simulink model "systeme_complet"  (R2022b)
settings: Solver=FixedStepAuto  StartTime=0.0  StopTime=t_stop  FixedStep=Ts  RelTol=1e-3
InitFcn:
  | parametres
undefined symbols (not defined in the file): f_dec, f_out, I_ref, Ki, Kp, M_ref, R_ch, Ts
libraries: fl_lib x22, ee_lib x18, nesl_utility x17, simulink x2, slpidlib x1
settings Model: Creator=HP  LastModifiedBy=HP

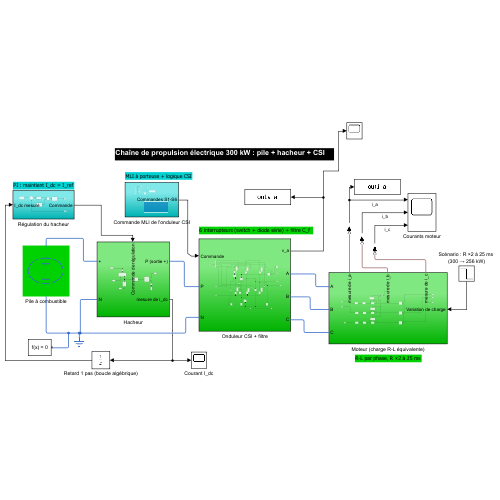
[thumbnail: Simulink's stored preview of the top-level diagram]
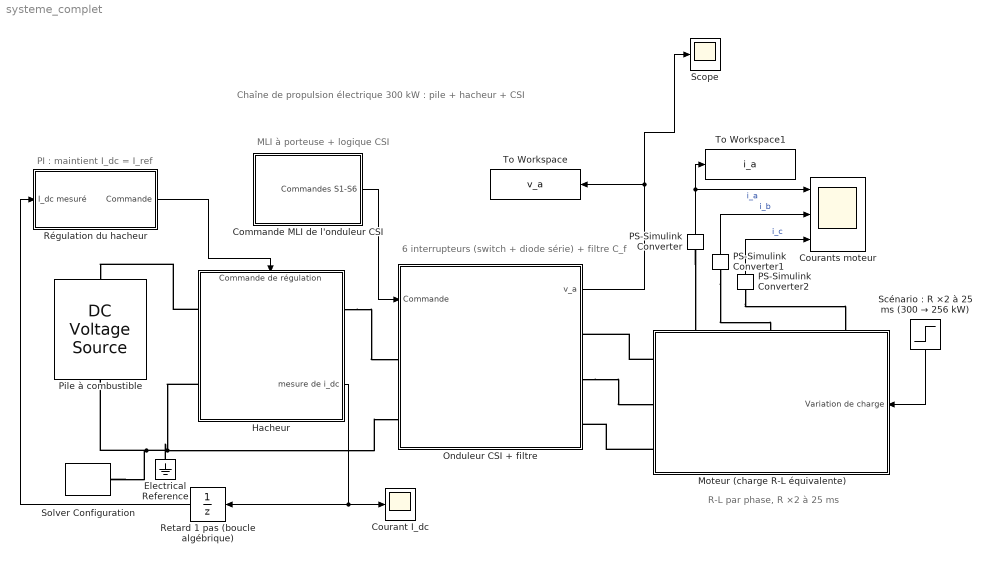
== system systeme_complet ==
  note: R-L par phase, R ×2 à 25 ms
  note: 6 interrupteurs (switch + diode série) + filtre C_f
  note: MLI à porteuse + logique CSI
  note: PI : maintient I_dc = I_ref
  note: Chaîne de propulsion électrique 300 kW : pile + hacheur + CSI
  Commande MLI de l'onduleur CSI : Subsystem
  Courant I_dc : Scope
  Courants moteur : Scope  NumInputPorts=3
  Electrical Reference : fl_lib/Electrical/Electrical Elements/Electrical Reference
  Hacheur : Subsystem
      settings: PortSchema="{\"entries\":[{\"content\":{\"sides\":[{\"content\":{\"connectorIds\":[\"LConn1\",\"LConn2\"]},\"type\":\"ConnectorPlacement.EquallySpacedRectSide\",\"uuid\":\"2dac1032-4ca4-4438-a519-692aa5ca1595\"},{\"content\":{\"connectorIds\":[\"RConn1\",\"Out1\"],\"side\":\"RIGHT\"},\"type\":\"ConnectorPlacement.EquallySpacedRectSide\",\"uuid\":\"94db1daf-747a-46bc-a51a-2b17978c1da3\"},{\"content\":{\"connectorIds\":[\"In1\"],\"side\":\"TOP\"},\"type\":\"ConnectorPlacement.EquallySpacedRectSide\",\"uuid\":\"3d1b3b24-76d5-4cf6-b9a4-916d1a1a4593\"},{\"content\":{\"connectorIds\":[],\"side\":\"BOTTOM\"},\"type\":\"ConnectorPlacement.EquallySpacedRectSide\",\"uuid\":\"3f80dfdd-caf6-41fc-aca6-59b801a18497\"}]},\"type\":\"ConnectorPlacement.EquallySpacedConnector\",\"uuid\":\"7bb300ac-b427-4bc8-9636-bf9acc93662d\"}],\"packageUris\":[\"http://schema.mathworks.com/mf0/Connector/R2020b\"],\"version\":\"1.0\"}"
  Moteur (charge R-L équivalente) : Subsystem
      settings: PortSchema="{\"entries\":[{\"content\":{\"sides\":[{\"content\":{\"connectorIds\":[\"LConn1\",\"LConn2\",\"LConn3\"]},\"type\":\"ConnectorPlacement.EquallySpacedRectSide\",\"uuid\":\"3a5aebfa-ac8c-4dc1-bdc7-0f42fa247e71\"},{\"content\":{\"connectorIds\":[\"In1\"],\"side\":\"RIGHT\"},\"type\":\"ConnectorPlacement.EquallySpacedRectSide\",\"uuid\":\"61d8263a-5991-459d-931c-dea362971dfc\"},{\"content\":{\"connectorIds\":[\"LConn4\",\"LConn5\",\"LConn6\"],\"side\":\"TOP\"},\"type\":\"ConnectorPlacement.EquallySpacedRectSide\",\"uuid\":\"dbe65e42-3578-4df4-96b5-9b98adcff1b2\"}]},\"type\":\"ConnectorPlacement.EquallySpacedConnector\",\"uuid\":\"a1fde088-52d3-4f5b-92ff-46a317a2fe9e\"}],\"packageUris\":[\"http://schema.mathworks.com/mf0/Connector/R2020b\"],\"version\":\"1.0\"}"
  Onduleur CSI + filtre : Subsystem
  PS-Simulink Converter : nesl_utility/PS-Simulink Converter  PhysicalDomain=network_engine_domain  SubClassName=ps_output  LeftPortType=input  RightPortType=output  PseudoPeriodic=off  Frequencies=[]  VectorFormat=inherit  Unit=A  AffineConversion=off
  PS-Simulink Converter1 : nesl_utility/PS-Simulink Converter  PhysicalDomain=network_engine_domain  SubClassName=ps_output  LeftPortType=input  RightPortType=output  PseudoPeriodic=off  Frequencies=[]  VectorFormat=inherit  Unit=A  AffineConversion=off
  PS-Simulink Converter2 : nesl_utility/PS-Simulink Converter  PhysicalDomain=network_engine_domain  SubClassName=ps_output  LeftPortType=input  RightPortType=output  PseudoPeriodic=off  Frequencies=[]  VectorFormat=inherit  Unit=A  AffineConversion=off
  Pile à combustible : fl_lib/Electrical/Electrical Sources/DC Voltage Source  v0=V_pile V
  Retard 1 pas (boucle algébrique) : UnitDelay  SampleTime=-1  HasFrameUpgradeWarning=on
  Régulation du hacheur : Subsystem
  Scope : Scope
  "Scénario : R ×2 à 25 ms (300 → 256 kW)" : Step  Time=0.025  Before=1  After=0  SampleTime=0
  Solver Configuration : nesl_utility/Solver Configuration  PhysicalDomain=network_engine_domain  SubClassName=solver  LeftPortType=input  RightPortType=generic  Tones=[]  Harmonics=[]  SimulateNoise=off  Profile=off  UseLocalSampling=off  EnableSwitchedLinearOptims=on  FrequencyDomain=off  UseCCode=off  RelTol=0.001  AbsTol=0.001  MinStep=1e-09  ToWorkspace=off  RevertToSquareIcSolve=off  NumHomotopyIterations=100  PhasorMode=off  PhasorModeNumHarmonics=1  ConsistencySolver=NEWTON_XTOL_AFTER_FTOL  IndexReductionMethod=DerivativeReplacement  DoDC=off  ResidualTolerance=1e-09  ConsistencyTolSource=GLOBAL  ConsistencyAbsTol=0.001  ConsistencyRelTol=0.001  ConsistencyTolFactor=0.001  UseLocalSolver=on  LocalSolverChoice=NE_PARTITIONING_ADVANCER  ResolveIndetEquations=on  FunctionEvalNumThread=1  LocalSolverSampleTime=Ts  DoFixedCost=on  MaxNonlinIter=3  MaxModeIter=2  ComputeImpulses=off  ImpulseIterations=2  LinearAlgebra=auto  LinearAlgebraNumThread=0  EquationFormulation=NE_TIME_EF  DelaysMemoryBudget=1024  AutomaticFiltering=on  FilteringTimeConstant=0.001  PartitionStorageMethod=AS_NEEDED  PartitionMemoryBudget=1024  PartitionMethod=ROBUST
  To Workspace : ToWorkspace  VariableName=v_a  SaveFormat=Timeseries  SampleTime=Ts
  To Workspace1 : ToWorkspace  VariableName=i_a  SaveFormat=Timeseries  SampleTime=Ts
  wires:
  PS-Simulink Converter/1 -> Courants moteur/1, To Workspace1/1  "i_a"
  PS-Simulink Converter1/1 -> Courants moteur/2  "i_b"
  PS-Simulink Converter2/1 -> Courants moteur/3  "i_c"
  Hacheur/1(mesure de i_dc) -> Retard 1 pas (boucle algébrique)/1, Courant I_dc/1
  "Scénario : R ×2 à 25 ms (300 → 256 kW)"/1 -> Moteur (charge R-L équivalente)/1(Variation de charge)
  Retard 1 pas (boucle algébrique)/1 -> Régulation du hacheur/1(I_dc mesuré)
  Régulation du hacheur/1(Commande) -> Hacheur/1(Commande de régulation)
  Commande MLI de l'onduleur CSI/1(Commandes S1-S6) -> Onduleur CSI + filtre/1(Commande)
  Onduleur CSI + filtre/1(v_a) -> Scope/1, To Workspace/1
  connections:
  Hacheur/LConn1 -- Pile à combustible/LConn1
  Hacheur/LConn2 -- Electrical Reference/LConn1 -- Pile à combustible/RConn1 -- Solver Configuration/RConn1 -- Onduleur CSI + filtre/LConn2
  PS-Simulink Converter/LConn1 -- Moteur (charge R-L équivalente)/LConn4
  PS-Simulink Converter1/LConn1 -- Moteur (charge R-L équivalente)/LConn5
  PS-Simulink Converter2/LConn1 -- Moteur (charge R-L équivalente)/LConn6
  Hacheur/RConn1 -- Onduleur CSI + filtre/LConn1
  Moteur (charge R-L équivalente)/LConn3 -- Onduleur CSI + filtre/RConn3
  Moteur (charge R-L équivalente)/LConn1 -- Onduleur CSI + filtre/RConn1
  Onduleur CSI + filtre/RConn2 -- Moteur (charge R-L équivalente)/LConn2

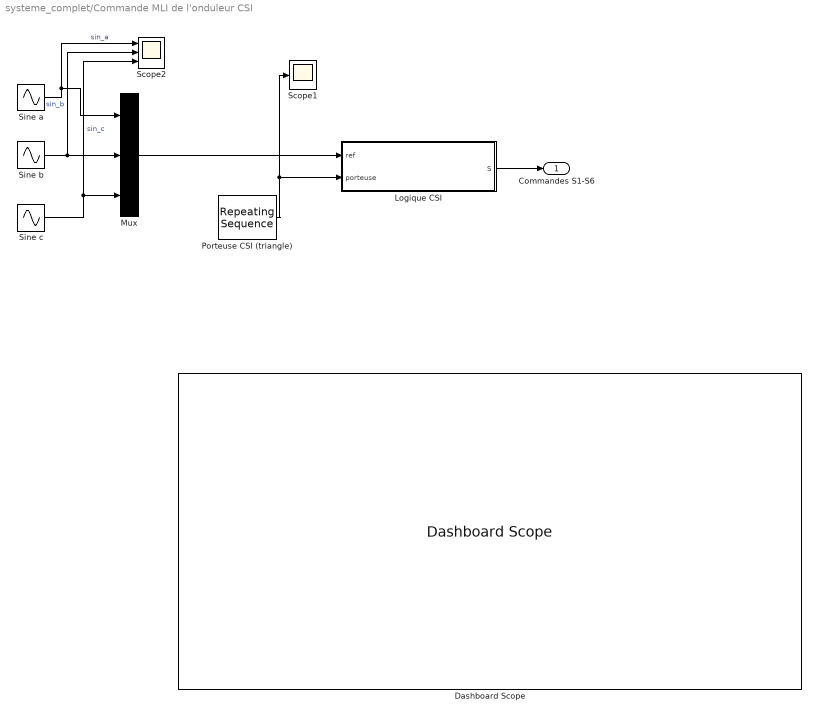
== system systeme_complet/Commande MLI de l'onduleur CSI ==
  Dashboard Scope : DashboardScope
  Logique CSI : MATLAB Function  TreatAsAtomicUnit=on
  Mux : Mux  Inputs=3
  Porteuse CSI (triangle) : simulink/Sources/Repeating Sequence  rep_seq_t=[0 1/(2*f_dec) 1/f_dec]  rep_seq_y=[-1 1 -1]
  Scope1 : Scope
  Scope2 : Scope  NumInputPorts=3
  Sine a : Sin  Amplitude=M_ref  Frequency=2*pi*f_out  SampleTime=Ts
  Sine b : Sin  Amplitude=M_ref  Frequency=2*pi*f_out  Phase=-2*pi/3  SampleTime=Ts
  Sine c : Sin  Amplitude=M_ref  Frequency=2*pi*f_out  Phase=2*pi/3  SampleTime=Ts
  Commandes S1-S6 : Outport
  wires:
  Logique CSI/1(S) -> Commandes S1-S6/1
  Sine b/1 -> Scope2/2, Mux/2  "sin_b"
  Sine c/1 -> Scope2/3, Mux/3  "sin_c"
  Mux/1 -> Logique CSI/1(ref)
  Sine a/1 -> Scope2/1, Mux/1  "sin_a"
  Porteuse CSI (triangle)/1 -> Scope1/1, Logique CSI/2(porteuse)

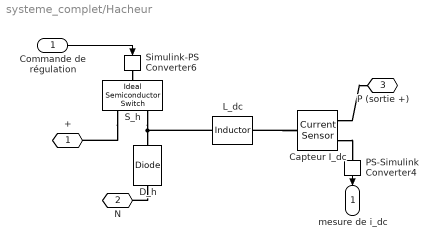
== system systeme_complet/Hacheur ==
  Commande de régulation : Inport
  Capteur I_dc : fl_lib/Electrical/Electrical Sensors/Current Sensor
  D_h : ee_lib/Semiconductors & Converters/Diode  ModelType=ee.enum.diode.modelType.pwl  TableType=ee.enum.diode.tableType.IfMat  IfMat=[.07, .12, .19, 1.75, 4.24, 7.32, 11.2; .16, .3, .72, 2.14, 5.02, 8.35, 13.12] A  VfMat=[.9, 1.15, 1.25, 1.5, 1.75, 2.17, 2.6, 2.85; .58, .68, .75, 1.1, 1.38, 1.77, 2.27, 2.7] V  TjVec=[25, 125] degC  VfVec=[.5, .7, .9, 1.3, 1.7, 2.1, 2.5] V  IfVec=[.1, .2, .5, 1, 2, 4, 7, 10] A  Vf=V_f V  Ron=R_on Ohm  Goff=G_off S  prmExp=ee.enum.diode.expParam.useTwo  I12=[.0137, .545] A  V12=[.6, .7] V  RS=0 Ohm  Tmeas=25 degC  IS=1e-12 A  ec=1  I1=0.0137 A  V1=0.6 V  N_series=1  N_parallel=1  Rz=0.3 Ohm  BV=inf V  C_param=ee.enum.diode.capParam.fixed  CJ=0 pF  CJ0=5 pF  Vvec=[.1, 10, 100] V  Cvec=[3.5, 1, .4] pF  VJ=1 V  Mgrad=0.5  FC=0.5  Q_param=ee.enum.diode.recoveryParam.off  iRM=-7.15 A  iF=4 A  didt=-750 A/us  trr_factor=3  trr=115 ns  Qrr=150 nA*s  Vr=-600 V  Ls=150 nH  Erec=0.03 J  TT=50 ns  tau=100 ns  T_param=ee.enum.diode.temperatureParam.off  Tdevice=25 degC  I1_T2=0.245 A  V1_T2=0.5 V  IS_T2=1.25e-7 A  Tmeas2=125 degC  XTI_param=ee.enum.diode.xtiParam.pn  XTI=3  EG_param=ee.enum.diode.egapParam.material_si  EG=1.11 eV  dBVdT=0 V/K  enable_faults=simscape.enum.onoff.off  fault_action=simscape.enum.assert.action.none  fault_types=ee.enum.diode.faults.open  tau_fault=1e-3 s  IfMat_faulted=[.07, .12, .19, 1.75, 4.24, 7.32, 11.2; .16, .3, .72, 2.14, 4.02, 6.35, 9.12] A  VfMat_faulted=[.9, 1.15, 1.25, 1.5, 1.75, 2.17, 2.6, 2.85; .58, .68, .75, 1.1, 1.38, 1.77, 2.27, 2.7] V  VfVec_faulted=[.5, .7, .9, 1.3, 1.7, 2.1, 2.5] V  IfVec_faulted=[.1, .2, .5, 1, 2, 4, 7, 10] A  Ropen_faulted=1000 Ohm  Gshort_faulted=1000 1/Ohm  Vf_faulted=0.6 V  Ron_faulted=0.3 Ohm  Goff_faulted=1e-8 S  I12_faulted=[.0137, .545] A  V12_faulted=[.6, .7] V  IS_faulted=1e-12 A  ec_faulted=1  I1_faulted=0.0137 A  V1_faulted=0.6 V  RS_faulted=0 Ohm  Rz_faulted=0.3 Ohm  BV_faulted=inf V  Cscale_faulted=100  enable_temporal_fault=simscape.enum.onoff.off  t_fault=inf s  enable_behavioral_fault=simscape.enum.onoff.off  max_permissible_voltage=inf V  n_fail_on_voltage=1  max_permissible_current=inf A  t_fail_on_current=1 s  max_permissible_dVdt=inf V/s  enable_fault_input=simscape.enum.onoff.off  i_specify=off  i_priority=None  i=0 A  i_nominal_specify=off  i_nominal_unit=A  i_nominal_value=1  v_specify=off  v_priority=None  v=0 V  v_nominal_specify=off  v_nominal_unit=V  v_nominal_value=1  v_capacitor_specify=off  v_capacitor_priority=None  v_capacitor=0 V  v_capacitor_nominal_specify=off  v_capacitor_nominal_unit=V  v_capacitor_nominal_value=1  i_diode_specify=off  i_diode_priority=None  i_diode=0 A  i_diode_nominal_specify=off  i_diode_nominal_unit=A  i_diode_nominal_value=1  v_diode_specify=off  v_diode_priority=None  v_diode=0 V  v_diode_nominal_specify=off  v_diode_nominal_unit=V  v_diode_nominal_value=1  i_capacitor_specify=off  i_capacitor_priority=None  i_capacitor=0 A  i_capacitor_nominal_specify=off  i_capacitor_nominal_unit=A  i_capacitor_nominal_value=1  power_dissipated_specify=off  power_dissipated_priority=None  power_dissipated=0 W  power_dissipated_nominal_specify=off  power_dissipated_nominal_unit=W  power_dissipated_nominal_value=1  fidelity_level=ee.enum.diode.fidelity.includeChargeDyn  rec_loss_model=ee.enum.diode.reverseRecoveryModel.fixed  ErecVal=0 J  ErecMat=zeros(2, 3) J  TjrecVec=[298.15, 398.15] K  IfrecVec=[.1, 1, 10] A  VrecVal=10 V  tFilter=1 / 1000 / 100 s  max_permissible_temperature=inf K  t_fail_on_temperature=1 s  thermal_network_parameterization=ee.enum.thermalNetworkTopology.junctionCase  Rth=[0, 10] K/W  Rth_Cauer=[1, 3, 10] K/W  Rth_Foster=[4, 6] K/W  thermal_mass_parameterization=ee.enum.thermalNetwork.timeconstant  thermal_mass=[0, 1] J/K  thermal_mass_Cauer=[.1, .3, 1] J/K  thermal_mass_Foster=[1.5, 3] J/K  thermal_time_constant=[0, 10] s  thermal_time_constant_Cauer=[1, 3, 10] s  thermal_time_constant_Foster=[6, 18] s  thermal_mass_initial_temperatures=[25, 25] degC  thermal_mass_initial_temperatures_Cauer=[25, 25, 25] degC  junction_thermal_mass=0.01 J/K  Tvec_initial_Foster=[25, 25, 25, 25] degC  no_thermal_network=0  junction_temperature_specify=off  junction_temperature_priority=None  junction_temperature=25 degC  junction_temperature_nominal_specify=off  junction_temperature_nominal_unit=degC  junction_temperature_nominal_value=1
  L_dc : ee_lib/Passive/Inductor  l=L_dc H  enable_L_tol=0  L_tol=20  tol_distribution=1  nSigma=4  r=0 Ohm  g=1e-9 1/Ohm  enable_operating_limits=0  operating_limit_action=2  max_working_current=1 A  power_rating=1 W  enable_faults=0  fault_action=1  lambdaPercent=50  k_faulted=0.9999  turnsShort=0  openCct=0  groundShort=0  groundShortG=0 1/Ohm  tau_fault=1e-3 s  enable_temporal_fault=0  t_fault=1 s  enable_behavioral_fault=0  max_permissible_voltage=100 V  n_fail_on_voltage=1  max_permissible_current=1 A  t_fail_on_current=1 s  i_L_specify=off  i_L_priority=High  i_L=0 A  i_L_nominal_specify=off  i_L_nominal_unit=A  i_L_nominal_value=1
  PS-Simulink Converter4 : nesl_utility/PS-Simulink Converter  PhysicalDomain=network_engine_domain  SubClassName=ps_output  LeftPortType=input  RightPortType=output  PseudoPeriodic=off  Frequencies=[]  VectorFormat=inherit  Unit=A  AffineConversion=off
  S_h : ee_lib/Semiconductors & Converters/Ideal Semiconductor Switch  port_option=ee.enum.controlport.ps  Ron=R_on Ohm  Goff=G_off 1/Ohm  Vth=0.5 V  diode_param=ee.enum.converters.protectiondiode.none  diode_Vf=0.8 V  diode_Ron=0.001 Ohm  diode_Goff=1e-5 1/Ohm  diode_C=50e-9 F  diode_iRM=-235 A  diode_iF=300 A  diode_idot=-50 A/us  diode_trr_param=ee.enum.converters.diodetrr.trr_factor  diode_trr_factor=3  diode_trr=15 us  diode_Qrr=1500 s*uA
  Simulink-PS Converter6 : nesl_utility/Simulink-PS Converter  PhysicalDomain=network_engine_domain  SubClassName=ps_input  LeftPortType=input  RightPortType=output  PseudoPeriodic=off  Frequencies=[]  NoiseDistribution=none  NoiseParameters=[]  Unit=1  AffineConversion=off  FilteringAndDerivatives=provide  SimscapeFilterOrder=1  InputFilterTimeConstant=0.001  UdotUserProvided=0
  + : PMIOPort  Side=Left
  N : PMIOPort  Port=2  Side=Left
  P (sortie +) : PMIOPort  Port=3  Side=Right
  mesure de i_dc : Outport
  wires:
  Commande de régulation/1 -> Simulink-PS Converter6/1
  PS-Simulink Converter4/1 -> mesure de i_dc/1
  connections:
  Capteur I_dc/LConn1 -- L_dc/RConn1
  Simulink-PS Converter6/RConn1 -- S_h/LConn1
  D_h/RConn1 -- S_h/RConn2 -- L_dc/LConn1
  S_h/RConn1 -- +/RConn1
  Capteur I_dc/RConn1 -- PS-Simulink Converter4/LConn1
  Capteur I_dc/RConn2 -- P (sortie +)/RConn1
  D_h/LConn1 -- N/RConn1

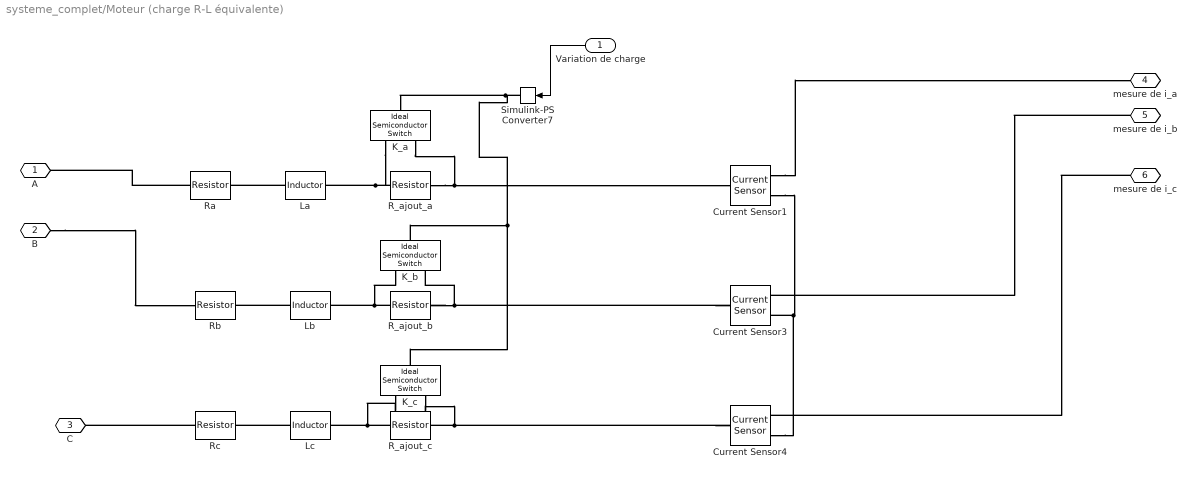
== system systeme_complet/Moteur (charge R-L équivalente) ==
  Variation de charge : Inport
  Current Sensor1 : fl_lib/Electrical/Electrical Sensors/Current Sensor
  Current Sensor3 : fl_lib/Electrical/Electrical Sensors/Current Sensor
  Current Sensor4 : fl_lib/Electrical/Electrical Sensors/Current Sensor
  K_a : ee_lib/Semiconductors & Converters/Ideal Semiconductor Switch  port_option=ee.enum.controlport.ps  Ron=R_on Ohm  Goff=G_off 1/Ohm  Vth=0.5 V  diode_param=ee.enum.converters.protectiondiode.none  diode_Vf=0.8 V  diode_Ron=0.001 Ohm  diode_Goff=1e-5 1/Ohm  diode_C=50e-9 F  diode_iRM=-235 A  diode_iF=300 A  diode_idot=-50 A/us  diode_trr_param=ee.enum.converters.diodetrr.trr_factor  diode_trr_factor=3  diode_trr=15 us  diode_Qrr=1500 s*uA
  K_b : ee_lib/Semiconductors & Converters/Ideal Semiconductor Switch  port_option=ee.enum.controlport.ps  Ron=R_on Ohm  Goff=G_off 1/Ohm  Vth=0.5 V  diode_param=ee.enum.converters.protectiondiode.none  diode_Vf=0.8 V  diode_Ron=0.001 Ohm  diode_Goff=1e-5 1/Ohm  diode_C=50e-9 F  diode_iRM=-235 A  diode_iF=300 A  diode_idot=-50 A/us  diode_trr_param=ee.enum.converters.diodetrr.trr_factor  diode_trr_factor=3  diode_trr=15 us  diode_Qrr=1500 s*uA
  K_c : ee_lib/Semiconductors & Converters/Ideal Semiconductor Switch  port_option=ee.enum.controlport.ps  Ron=R_on Ohm  Goff=G_off 1/Ohm  Vth=0.5 V  diode_param=ee.enum.converters.protectiondiode.none  diode_Vf=0.8 V  diode_Ron=0.001 Ohm  diode_Goff=1e-5 1/Ohm  diode_C=50e-9 F  diode_iRM=-235 A  diode_iF=300 A  diode_idot=-50 A/us  diode_trr_param=ee.enum.converters.diodetrr.trr_factor  diode_trr_factor=3  diode_trr=15 us  diode_Qrr=1500 s*uA
  La : fl_lib/Electrical/Electrical Elements/Inductor  l=L_ch H  r=0 Ohm  g=1e-9 1/Ohm  i_specify=off  i_priority=None  i=0 A  i_nominal_specify=off  i_nominal_unit=A  i_nominal_value=1  v_specify=off  v_priority=None  v=0 V  v_nominal_specify=off  v_nominal_unit=V  v_nominal_value=1  i_L_specify=off  i_L_priority=High  i_L=0 A  i_L_nominal_specify=off  i_L_nominal_unit=A  i_L_nominal_value=1
  Lb : fl_lib/Electrical/Electrical Elements/Inductor  l=L_ch H  r=0 Ohm  g=1e-9 1/Ohm  i_specify=off  i_priority=None  i=0 A  i_nominal_specify=off  i_nominal_unit=A  i_nominal_value=1  v_specify=off  v_priority=None  v=0 V  v_nominal_specify=off  v_nominal_unit=V  v_nominal_value=1  i_L_specify=off  i_L_priority=High  i_L=0 A  i_L_nominal_specify=off  i_L_nominal_unit=A  i_L_nominal_value=1
  Lc : fl_lib/Electrical/Electrical Elements/Inductor  l=L_ch H  r=0 Ohm  g=1e-9 1/Ohm  i_specify=off  i_priority=None  i=0 A  i_nominal_specify=off  i_nominal_unit=A  i_nominal_value=1  v_specify=off  v_priority=None  v=0 V  v_nominal_specify=off  v_nominal_unit=V  v_nominal_value=1  i_L_specify=off  i_L_priority=High  i_L=0 A  i_L_nominal_specify=off  i_L_nominal_unit=A  i_L_nominal_value=1
  R_ajout_a : fl_lib/Electrical/Electrical Elements/Resistor  R=R_ch Ohm  i_specify=off  i_priority=None  i=0 A  i_nominal_specify=off  i_nominal_unit=A  i_nominal_value=1  v_specify=off  v_priority=None  v=0 V  v_nominal_specify=off  v_nominal_unit=V  v_nominal_value=1
  R_ajout_b : fl_lib/Electrical/Electrical Elements/Resistor  R=R_ch Ohm  i_specify=off  i_priority=None  i=0 A  i_nominal_specify=off  i_nominal_unit=A  i_nominal_value=1  v_specify=off  v_priority=None  v=0 V  v_nominal_specify=off  v_nominal_unit=V  v_nominal_value=1
  R_ajout_c : fl_lib/Electrical/Electrical Elements/Resistor  R=R_ch Ohm  i_specify=off  i_priority=None  i=0 A  i_nominal_specify=off  i_nominal_unit=A  i_nominal_value=1  v_specify=off  v_priority=None  v=0 V  v_nominal_specify=off  v_nominal_unit=V  v_nominal_value=1
  Ra : fl_lib/Electrical/Electrical Elements/Resistor  R=R_ch Ohm  i_specify=off  i_priority=None  i=0 A  i_nominal_specify=off  i_nominal_unit=A  i_nominal_value=1  v_specify=off  v_priority=None  v=0 V  v_nominal_specify=off  v_nominal_unit=V  v_nominal_value=1
  Rb : fl_lib/Electrical/Electrical Elements/Resistor  R=R_ch Ohm  i_specify=off  i_priority=None  i=0 A  i_nominal_specify=off  i_nominal_unit=A  i_nominal_value=1  v_specify=off  v_priority=None  v=0 V  v_nominal_specify=off  v_nominal_unit=V  v_nominal_value=1
  Rc : fl_lib/Electrical/Electrical Elements/Resistor  R=R_ch Ohm  i_specify=off  i_priority=None  i=0 A  i_nominal_specify=off  i_nominal_unit=A  i_nominal_value=1  v_specify=off  v_priority=None  v=0 V  v_nominal_specify=off  v_nominal_unit=V  v_nominal_value=1
  Simulink-PS Converter7 : nesl_utility/Simulink-PS Converter  PhysicalDomain=network_engine_domain  SubClassName=ps_input  LeftPortType=input  RightPortType=output  PseudoPeriodic=off  Frequencies=[]  NoiseDistribution=none  NoiseParameters=[]  Unit=1  AffineConversion=off  FilteringAndDerivatives=provide  SimscapeFilterOrder=1  InputFilterTimeConstant=0.001  UdotUserProvided=0
  A : PMIOPort  Side=Left
  B : PMIOPort  Port=2  Side=Left
  C : PMIOPort  Port=3  Side=Left
  mesure de i_a : PMIOPort  Port=4  Side=Left
  mesure de i_b : PMIOPort  Port=5  Side=Left
  mesure de i_c : PMIOPort  Port=6  Side=Left
  wires:
  Variation de charge/1 -> Simulink-PS Converter7/1
  connections:
  Lb/LConn1 -- Rb/RConn1
  Simulink-PS Converter7/RConn1 -- K_c/LConn1 -- K_b/LConn1 -- K_a/LConn1
  R_ajout_b/LConn1 -- Lb/RConn1 -- K_b/RConn1
  Lc/LConn1 -- Rc/RConn1
  La/LConn1 -- Ra/RConn1
  Ra/LConn1 -- A/RConn1
  Rc/LConn1 -- C/RConn1
  R_ajout_a/LConn1 -- La/RConn1 -- K_a/RConn1
  R_ajout_c/LConn1 -- K_c/RConn1 -- Lc/RConn1
  B/RConn1 -- Rb/LConn1
  Current Sensor1/RConn1 -- mesure de i_a/RConn1
  mesure de i_b/RConn1 -- Current Sensor3/RConn1
  Current Sensor1/RConn2 -- Current Sensor4/RConn2 -- Current Sensor3/RConn2
  mesure de i_c/RConn1 -- Current Sensor4/RConn1
  R_ajout_a/RConn1 -- K_a/RConn2 -- Current Sensor1/LConn1
  Current Sensor4/LConn1 -- K_c/RConn2 -- R_ajout_c/RConn1
  Current Sensor3/LConn1 -- R_ajout_b/RConn1 -- K_b/RConn2

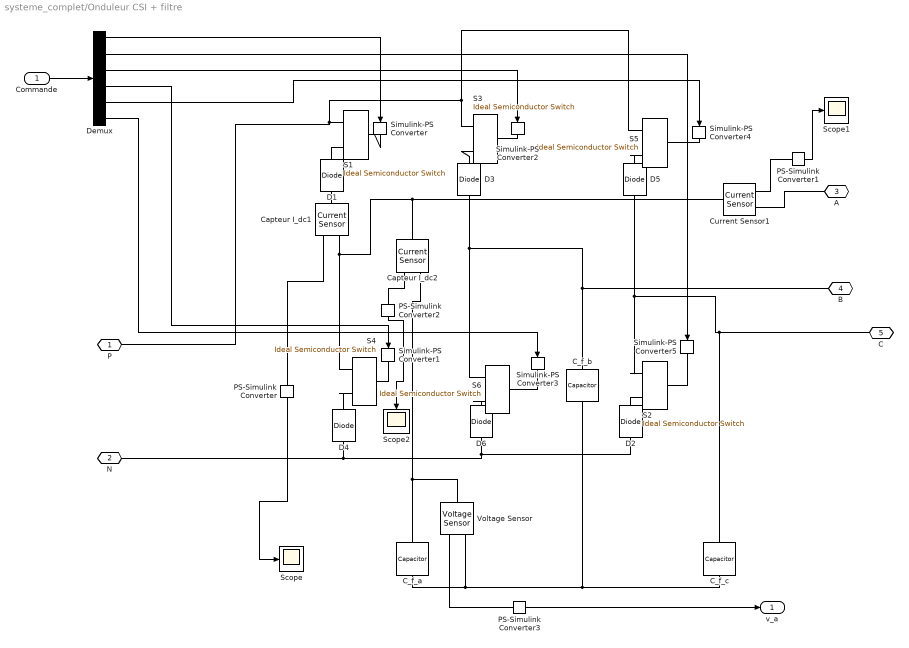
== system systeme_complet/Onduleur CSI + filtre ==
  Commande : Inport
  C_f_a : fl_lib/Electrical/Electrical Elements/Capacitor  c=C_f F  r=1e-6 Ohm  g=0 1/Ohm  i_specify=off  i_priority=None  i=0 A  i_nominal_specify=off  i_nominal_unit=A  i_nominal_value=1  v_specify=off  v_priority=None  v=0 V  v_nominal_specify=off  v_nominal_unit=V  v_nominal_value=1  vc_specify=off  vc_priority=High  vc=0 V  vc_nominal_specify=off  vc_nominal_unit=V  vc_nominal_value=1
  C_f_b : fl_lib/Electrical/Electrical Elements/Capacitor  c=C_f F  r=1e-6 Ohm  g=0 1/Ohm  i_specify=off  i_priority=None  i=0 A  i_nominal_specify=off  i_nominal_unit=A  i_nominal_value=1  v_specify=off  v_priority=None  v=0 V  v_nominal_specify=off  v_nominal_unit=V  v_nominal_value=1  vc_specify=off  vc_priority=High  vc=0 V  vc_nominal_specify=off  vc_nominal_unit=V  vc_nominal_value=1
  C_f_c : fl_lib/Electrical/Electrical Elements/Capacitor  c=C_f F  r=1e-6 Ohm  g=0 1/Ohm  i_specify=off  i_priority=None  i=0 A  i_nominal_specify=off  i_nominal_unit=A  i_nominal_value=1  v_specify=off  v_priority=None  v=0 V  v_nominal_specify=off  v_nominal_unit=V  v_nominal_value=1  vc_specify=off  vc_priority=High  vc=0 V  vc_nominal_specify=off  vc_nominal_unit=V  vc_nominal_value=1
  Capteur I_dc1 : fl_lib/Electrical/Electrical Sensors/Current Sensor
  Capteur I_dc2 : fl_lib/Electrical/Electrical Sensors/Current Sensor
  Current Sensor1 : fl_lib/Electrical/Electrical Sensors/Current Sensor
  D{1..6} (6 alike) : ee_lib/Semiconductors & Converters/Diode  ModelType=ee.enum.diode.modelType.pwl  TableType=ee.enum.diode.tableType.IfMat  IfMat=[.07, .12, .19, 1.75, 4.24, 7.32, 11.2; .16, .3, .72, 2.14, 5.02, 8.35, 13.12] A  VfMat=[.9, 1.15, 1.25, 1.5, 1.75, 2.17, 2.6, 2.85; .58, .68, .75, 1.1, 1.38, 1.77, 2.27, 2.7] V  TjVec=[25, 125] degC  VfVec=[.5, .7, .9, 1.3, 1.7, 2.1, 2.5] V  IfVec=[.1, .2, .5, 1, 2, 4, 7, 10] A  Vf=V_f V  Ron=R_on Ohm  Goff=G_off S  prmExp=ee.enum.diode.expParam.useTwo  I12=[.0137, .545] A  V12=[.6, .7] V  RS=0 Ohm  Tmeas=25 degC  IS=1e-12 A  ec=1  I1=0.0137 A  V1=0.6 V  N_series=1  N_parallel=1  Rz=0.3 Ohm  BV=inf V  C_param=ee.enum.diode.capParam.fixed  CJ=0 pF  CJ0=5 pF  Vvec=[.1, 10, 100] V  Cvec=[3.5, 1, .4] pF  VJ=1 V  Mgrad=0.5  FC=0.5  Q_param=ee.enum.diode.recoveryParam.off  iRM=-7.15 A  iF=4 A  didt=-750 A/us  trr_factor=3  trr=115 ns  Qrr=150 nA*s  Vr=-600 V  Ls=150 nH  Erec=0.03 J  TT=50 ns  tau=100 ns  T_param=ee.enum.diode.temperatureParam.off  Tdevice=25 degC  I1_T2=0.245 A  V1_T2=0.5 V  IS_T2=1.25e-7 A  Tmeas2=125 degC  XTI_param=ee.enum.diode.xtiParam.pn  XTI=3  EG_param=ee.enum.diode.egapParam.material_si  EG=1.11 eV  dBVdT=0 V/K  enable_faults=simscape.enum.onoff.off  fault_action=simscape.enum.assert.action.none  fault_types=ee.enum.diode.faults.open  tau_fault=1e-3 s  IfMat_faulted=[.07, .12, .19, 1.75, 4.24, 7.32, 11.2; .16, .3, .72, 2.14, 4.02, 6.35, 9.12] A  VfMat_faulted=[.9, 1.15, 1.25, 1.5, 1.75, 2.17, 2.6, 2.85; .58, .68, .75, 1.1, 1.38, 1.77, 2.27, 2.7] V  VfVec_faulted=[.5, .7, .9, 1.3, 1.7, 2.1, 2.5] V  IfVec_faulted=[.1, .2, .5, 1, 2, 4, 7, 10] A  Ropen_faulted=1000 Ohm  Gshort_faulted=1000 1/Ohm  Vf_faulted=0.6 V  Ron_faulted=0.3 Ohm  Goff_faulted=1e-8 S  I12_faulted=[.0137, .545] A  V12_faulted=[.6, .7] V  IS_faulted=1e-12 A  ec_faulted=1  I1_faulted=0.0137 A  V1_faulted=0.6 V  RS_faulted=0 Ohm  Rz_faulted=0.3 Ohm  BV_faulted=inf V  Cscale_faulted=100  enable_temporal_fault=simscape.enum.onoff.off  t_fault=inf s  enable_behavioral_fault=simscape.enum.onoff.off  max_permissible_voltage=inf V  n_fail_on_voltage=1  max_permissible_current=inf A  t_fail_on_current=1 s  max_permissible_dVdt=inf V/s  enable_fault_input=simscape.enum.onoff.off  i_specify=off  i_priority=None  i=0 A  i_nominal_specify=off  i_nominal_unit=A  i_nominal_value=1  v_specify=off  v_priority=None  v=0 V  v_nominal_specify=off  v_nominal_unit=V  v_nominal_value=1  v_capacitor_specify=off  v_capacitor_priority=None  v_capacitor=0 V  v_capacitor_nominal_specify=off  v_capacitor_nominal_unit=V  v_capacitor_nominal_value=1  i_diode_specify=off  i_diode_priority=None  i_diode=0 A  i_diode_nominal_specify=off  i_diode_nominal_unit=A  i_diode_nominal_value=1  v_diode_specify=off  v_diode_priority=None  v_diode=0 V  v_diode_nominal_specify=off  v_diode_nominal_unit=V  v_diode_nominal_value=1  i_capacitor_specify=off  i_capacitor_priority=None  i_capacitor=0 A  i_capacitor_nominal_specify=off  i_capacitor_nominal_unit=A  i_capacitor_nominal_value=1  power_dissipated_specify=off  power_dissipated_priority=None  power_dissipated=0 W  power_dissipated_nominal_specify=off  power_dissipated_nominal_unit=W  power_dissipated_nominal_value=1  fidelity_level=ee.enum.diode.fidelity.includeChargeDyn  rec_loss_model=ee.enum.diode.reverseRecoveryModel.fixed  ErecVal=0 J  ErecMat=zeros(2, 3) J  TjrecVec=[298.15, 398.15] K  IfrecVec=[.1, 1, 10] A  VrecVal=10 V  tFilter=1 / 1000 / 100 s  max_permissible_temperature=inf K  t_fail_on_temperature=1 s  thermal_network_parameterization=ee.enum.thermalNetworkTopology.junctionCase  Rth=[0, 10] K/W  Rth_Cauer=[1, 3, 10] K/W  Rth_Foster=[4, 6] K/W  thermal_mass_parameterization=ee.enum.thermalNetwork.timeconstant  thermal_mass=[0, 1] J/K  thermal_mass_Cauer=[.1, .3, 1] J/K  thermal_mass_Foster=[1.5, 3] J/K  thermal_time_constant=[0, 10] s  thermal_time_constant_Cauer=[1, 3, 10] s  thermal_time_constant_Foster=[6, 18] s  thermal_mass_initial_temperatures=[25, 25] degC  thermal_mass_initial_temperatures_Cauer=[25, 25, 25] degC  junction_thermal_mass=0.01 J/K  Tvec_initial_Foster=[25, 25, 25, 25] degC  no_thermal_network=0  junction_temperature_specify=off  junction_temperature_priority=None  junction_temperature=25 degC  junction_temperature_nominal_specify=off  junction_temperature_nominal_unit=degC  junction_temperature_nominal_value=1
  Demux : Demux  Outputs=6
  PS-Simulink Converter : nesl_utility/PS-Simulink Converter  PhysicalDomain=network_engine_domain  SubClassName=ps_output  LeftPortType=input  RightPortType=output  PseudoPeriodic=off  Frequencies=[]  VectorFormat=inherit  Unit=inherit  AffineConversion=off
  PS-Simulink Converter1 : nesl_utility/PS-Simulink Converter  PhysicalDomain=network_engine_domain  SubClassName=ps_output  LeftPortType=input  RightPortType=output  PseudoPeriodic=off  Frequencies=[]  VectorFormat=inherit  Unit=A  AffineConversion=off
  PS-Simulink Converter2 : nesl_utility/PS-Simulink Converter  PhysicalDomain=network_engine_domain  SubClassName=ps_output  LeftPortType=input  RightPortType=output  PseudoPeriodic=off  Frequencies=[]  VectorFormat=inherit  Unit=inherit  AffineConversion=off
  PS-Simulink Converter3 : nesl_utility/PS-Simulink Converter  PhysicalDomain=network_engine_domain  SubClassName=ps_output  LeftPortType=input  RightPortType=output  PseudoPeriodic=off  Frequencies=[]  VectorFormat=inherit  Unit=V  AffineConversion=off
  S{1..6} (6 alike) : ee_lib/Semiconductors & Converters/Ideal Semiconductor Switch  port_option=ee.enum.controlport.ps  Ron=R_on Ohm  Goff=G_off 1/Ohm  Vth=0.5 V  diode_param=ee.enum.converters.protectiondiode.none  diode_Vf=0.8 V  diode_Ron=0.001 Ohm  diode_Goff=1e-5 1/Ohm  diode_C=50e-9 F  diode_iRM=-235 A  diode_iF=300 A  diode_idot=-50 A/us  diode_trr_param=ee.enum.converters.diodetrr.trr_factor  diode_trr_factor=3  diode_trr=15 us  diode_Qrr=1500 s*uA
  Scope : Scope
  Scope1 : Scope
  Scope2 : Scope
  Simulink-PS Converter{,1..5} (6 alike) : nesl_utility/Simulink-PS Converter  PhysicalDomain=network_engine_domain  SubClassName=ps_input  LeftPortType=input  RightPortType=output  PseudoPeriodic=off  Frequencies=[]  NoiseDistribution=none  NoiseParameters=[]  Unit=1  AffineConversion=off  FilteringAndDerivatives=provide  SimscapeFilterOrder=1  InputFilterTimeConstant=0.001  UdotUserProvided=0
  Voltage Sensor : fl_lib/Electrical/Electrical Sensors/Voltage Sensor
  P : PMIOPort  Side=Left
  N : PMIOPort  Port=2  Side=Left
  A : PMIOPort  Port=3  Side=Right
  B : PMIOPort  Port=4  Side=Right
  C : PMIOPort  Port=5  Side=Right
  v_a : Outport
  wires:
  Demux/2 -> Simulink-PS Converter5/1
  Demux/4 -> Simulink-PS Converter1/1
  Demux/3 -> Simulink-PS Converter2/1
  Demux/1 -> Simulink-PS Converter/1
  Demux/6 -> Simulink-PS Converter3/1
  Demux/5 -> Simulink-PS Converter4/1
  PS-Simulink Converter3/1 -> v_a/1
  Commande/1 -> Demux/1
  PS-Simulink Converter/1 -> Scope/1
  PS-Simulink Converter1/1 -> Scope1/1
  PS-Simulink Converter2/1 -> Scope2/1
  connections:
  C_f_c/LConn1 -- C/RConn1 -- S2/RConn1 -- D5/RConn1
  S3/LConn1 -- Simulink-PS Converter2/RConn1
  C_f_b/LConn1 -- S6/RConn1 -- D3/RConn1 -- B/RConn1
  N/RConn1 -- D4/RConn1 -- D2/RConn1 -- D6/RConn1
  S4/RConn2 -- D4/LConn1
  S1/RConn1 -- P/RConn1 -- S5/RConn1 -- S3/RConn1
  S5/RConn2 -- D5/LConn1
  S6/RConn2 -- D6/LConn1
  C_f_b/RConn1 -- C_f_a/RConn1 -- Voltage Sensor/RConn2 -- C_f_c/RConn1
  S6/LConn1 -- Simulink-PS Converter3/RConn1
  S4/LConn1 -- Simulink-PS Converter1/RConn1
  S5/LConn1 -- Simulink-PS Converter4/RConn1
  Simulink-PS Converter/RConn1 -- S1/LConn1
  D1/LConn1 -- S1/RConn2
  S2/RConn2 -- D2/LConn1
  S2/LConn1 -- Simulink-PS Converter5/RConn1
  S3/RConn2 -- D3/LConn1
  PS-Simulink Converter3/LConn1 -- Voltage Sensor/RConn1
  A/RConn1 -- Current Sensor1/RConn2
  Current Sensor1/LConn1 -- Capteur I_dc2/LConn1 -- S4/RConn1 -- Capteur I_dc1/RConn2
  Capteur I_dc1/RConn1 -- PS-Simulink Converter/LConn1
  PS-Simulink Converter1/LConn1 -- Current Sensor1/RConn1
  Capteur I_dc1/LConn1 -- D1/RConn1
  PS-Simulink Converter2/LConn1 -- Capteur I_dc2/RConn1
  Capteur I_dc2/RConn2 -- Voltage Sensor/LConn1 -- C_f_a/LConn1

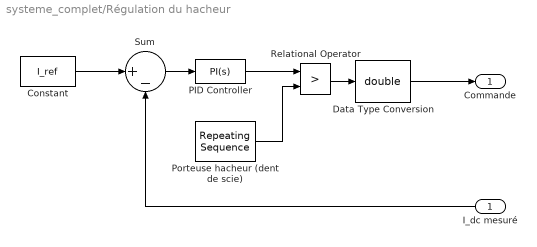
== system systeme_complet/Régulation du hacheur ==
  I_dc mesuré : Inport
  Constant : Constant  Value=I_ref
  Data Type Conversion : DataTypeConversion  OutDataTypeStr=double  SaturateOnIntegerOverflow=off  RndMeth=Floor
  PID Controller : slpidlib/PID Controller  Controller=PI  Form=Parallel  TimeDomain=Continuous-time  UseExternalTs=off  SampleTime=-1  IntegratorMethod=Forward Euler  FilterMethod=Forward Euler  ControllerParametersSource=internal  P=Kp  I=Ki  UseKiTs=off  D=0  N=100  UseFilter=on  TunerSelectOption=Transfer Function Based (PID Tuner App)  InitialConditionSource=internal  InitialConditionForIntegrator=0  InitialConditionForFilter=0  DifferentiatorICPrevScaledInput=0  ExternalReset=none  TrackingMode=off  Kt=1  LimitOutput=on  SatLimitsSource=internal  UpperSaturationLimit=0.95  LowerSaturationLimit=0  LinearizeAsGain=on  AntiWindupMode=clamping  Kb=1  LimitIntegrator=off  UpperIntegratorSaturationLimit=inf  LowerIntegratorSaturationLimit=-inf  POutMin=[]  POutMax=[]  IOutMin=[]  IOutMax=[]  DOutMin=[]  DOutMax=[]  NOutMin=[]  NOutMax=[]  SumOutMin=[]  SumOutMax=[]  SaturationOutMin=[]  SaturationOutMax=[]  PParamMin=[]  PParamMax=[]  IParamMin=[]  IParamMax=[]  DParamMin=[]  DParamMax=[]  NParamMin=[]  NParamMax=[]  KbParamMin=[]  KbParamMax=[]  KtParamMin=[]  KtParamMax=[]  KbOutMin=[]  KbOutMax=[]  KtOutMin=[]  KtOutMax=[]  IntegratorOutMin=[]  IntegratorOutMax=[]  FilterOutMin=[]  FilterOutMax=[]  SumI1OutMin=[]  SumI1OutMax=[]  SumI2OutMin=[]  SumI2OutMax=[]  SumI3OutMin=[]  SumI3OutMax=[]  SumI4OutMin=[]  SumI4OutMax=[]  SumDOutMin=[]  SumDOutMax=[]  DifferentiatorOutMin=[]  DifferentiatorOutMax=[]  FilterDiffOutCoefMin=[]  FilterDiffOutCoefMax=[]  ReciprocalOutMin=[]  ReciprocalOutMax=[]  SumDenOutMin=[]  SumDenOutMax=[]  SumNumOutMin=[]  SumNumOutMax=[]  DivideOutMin=[]  DivideOutMax=[]  UdiffTsProdOutMin=[]  UdiffTsProdOutMax=[]  NTsProdOutMin=[]  NTsProdOutMax=[]  UintegralTsProdOutMin=[]  UintegralTsProdOutMax=[]  UngainTsProdOutMin=[]  UngainTsProdOutMax=[]  ClampingZeroOutDataTypeStr=Inherit: Inherit via back propagation  ClampingZeroOutMin=[]  ClampingZeroOutMax=[]  FilterDenConstantOutDataTypeStr=Inherit: Inherit via back propagation  FilterDenConstantOutMin=[]  FilterDenConstantOutMax=[]  PCopyOutDataTypeStr=Inherit: Inherit via back propagation  PCopyOutMin=[]  PCopyOutMax=[]  NCopyOutDataTypeStr=Inherit: Inherit via back propagation  NCopyOutMin=[]  NCopyOutMax=[]  IntegratorContinuousStateAttributes=''  IntegratorStateMustResolveToSignalObject=off  IntegratorRTWStateStorageClass=Auto  FilterContinuousStateAttributes=''  FilterStateMustResolveToSignalObject=off  FilterRTWStateStorageClass=Auto  ParallelPVariant=InternalParameters  IdealPVariant=Disabled  IVariant=InternalParameters  DVariant=Disabled  IntegratorVariant=Continuous  SatVariant=Enabled  AWVariant=ContClampingParallel  PCopyVariant=Disabled  TRVariant=Disabled  FdbkBlocksVariant=Forward  IdealPFdbkVariant=Disabled  SatFdbkVariant=Disabled  DerivativeFilterVariant=Disabled  NVariant=Disabled  NCopyVariant=Disabled_SignalSpec  FilterICVariant=Disabled  IntegratorICVariant=InternalICs  ExternalResetVariant=Disabled  TRSumVariant=Passthrough  SumFdbkVariant=Disabled  SumVariant=Sum_PI  TsampFilterVariant=InternalTs  TsampNgainVariant=Passthrough  TsampIntegralVariant=Passthrough  ExternalSaturationOutDataTypeStr=Inherit: Same as second input
  Porteuse hacheur (dent de scie) : simulink/Sources/Repeating Sequence  rep_seq_t=[0 1/f_dec]  rep_seq_y=[0 1]
  Relational Operator : RelationalOperator  Operator=>  OutDataTypeStr=boolean  InputSameDT=off
  Sum : Sum  Inputs=|+-
  Commande : Outport
  wires:
  Porteuse hacheur (dent de scie)/1 -> Relational Operator/2
  Relational Operator/1 -> Data Type Conversion/1
  I_dc mesuré/1 -> Sum/2
  Data Type Conversion/1 -> Commande/1
  Sum/1 -> PID Controller/1
  PID Controller/1 -> Relational Operator/1
  Constant/1 -> Sum/1

== matlab function systeme_complet/Commande MLI de l'onduleur CSI/Logique CSI ==
  data: ref input; S output; porteuse input
function S = commande_csi(ref, porteuse)

    % ref      : les 3 sinusoïdes de référence (phases a, b, c)
    % porteuse : triangle entre -1 et 1 à f_dec
    % S        : commandes des interrupteurs [S1 S2 S3 S4 S5 S6]
    
    % Injection homopolaire : permet d'atteindre M_ref > 1
    v0 = -(max(ref) + min(ref))/2;
    r  = ref + v0;
    
    % Comparaison avec la porteuse (logique d'un onduleur de tension)
    g  = r > porteuse;
    ga = g(1); gb = g(2); gc = g(3);
    
    % État nul : les trois signaux sont égaux -> aucun chemin pour I_dc
    Z = (ga == gb) && (gb == gc);
    
    % Traduction vers le CSI : un interrupteur en haut, un en bas
    S = zeros(6,1);
    S(1) = (ga && ~gb) || Z;   % haut, phase a  (+ court-circuit si état nul)
    S(4) = (~ga && gb) || Z;   % bas,  phase a  (+ court-circuit si état nul)
    S(3) =  gb && ~gc;         % haut, phase b
    S(6) = ~gb &&  gc;         % bas,  phase b
    S(5) =  gc && ~ga;         % haut, phase c
    S(2) = ~gc &&  ga;         % bas,  phase c

end
